simulink model "MonumentSimulink"  (R2026a)
settings: Solver=VariableStepAuto  StopTime=24
libraries: fuzblock x1

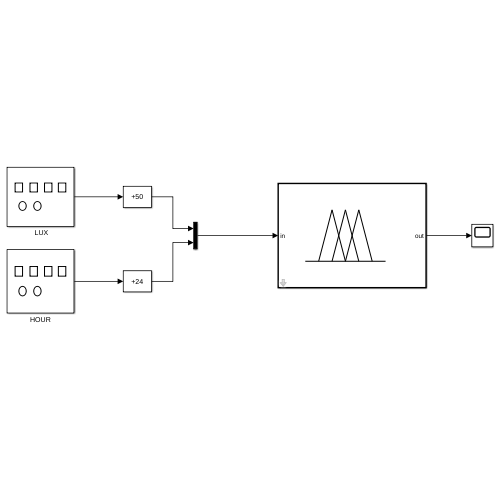
[thumbnail: Simulink's stored preview of the top-level diagram]
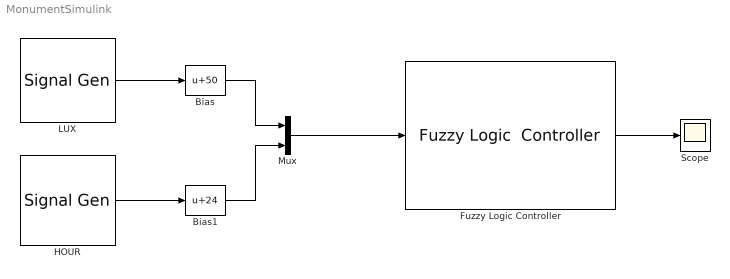
== system MonumentSimulink ==
  " LUX" : SignalGenerator  Amplitude=50  Frequency=0.05  Units=rad/sec
  Bias : Bias  Bias=50  SaturateOnIntegerOverflow=off
  Bias1 : Bias  Bias=24  SaturateOnIntegerOverflow=off
  Fuzzy Logic Controller : fuzblock/Fuzzy Logic  Controller  FIS=fis  OutputSampleNumber=101  DataType=double  UseLookupTable=off  NumBreakpoints=10  FuzzifiedInputs=off  RuleFiringStrengths=off  RuleOutputs=off  AggregatedOutputs=off  SimulateUsing=Interpreted execution  OutOfRangeInputValueMessage=warning  NoRuleFiredMessage=warning  EmptyOutputFuzzySetMessage=warning
  "HOUR " : SignalGenerator  Amplitude=6  Frequency=0.04  Units=rad/sec
  Mux : Mux  Inputs=2
  Scope : Scope
      settings: ActiveDisplayYMinimum=9.3049765765286612  ActiveDisplayYMaximum=54.521669269274611
  wires:
  Mux/1 -> Fuzzy Logic Controller/1
  Fuzzy Logic Controller/1 -> Scope/1
  " LUX"/1 -> Bias/1
  Bias/1 -> Mux/1
  "HOUR "/1 -> Bias1/1
  Bias1/1 -> Mux/2
